simulink library "Libs_second"  (R2023b)
settings: Solver=VariableStepAuto  StartTime=0.0  StopTime=10.0  RelTol=1e-3
libraries: $bdroot x3, simulink x1
(part 2 of 2)

== stateflow chart Libs_second/Node_N_V6/Automaton ==
  settings: updateMethod=DISCRETE  executeAtInitialization=1
  state PacemakerCell
    state Cell [parallel]
      settings: executionOrder=1
      state Slow
        en: q=1; %phase4
      state Stimulated
        en: q=2; %phase0
        f1theta=exp(-h*theta);
        Vmax=(-1)*MDP*f1theta;
        [f3theta,n,Vmin]=sat(n,hr,hs,Vh1,s,m,theta);
      state Plateau
        en: q=3;%phase2
      state RP
        en:q=0;%phase3
      (default) -> Slow : /{Vmin=0;Vmax=(-1)*MDP; d3=d3fcn(MDP,VR,VT,d0,d2,ERP); BCL=RR(BCLin,SDin,f1in,f2in,sigma1sqin,sigma2sqin,t);...
          | t3=(abs(MDP)-VR)/abs(d3); t0=VR/abs(d0);t2=(abs(MDP)-VT)/abs(d2);d1=(VT)/(BCL-t3-t0-t2);d1out=d1;}
      Slow -> Stimulated [order 1] : [gv>VT&& v<VT]{theta=(v-VT)/(Vmin-VT);f2theta=exp(-f*theta);d2out=d2*f2theta;...
          |  f4theta=exp(j*(theta-1)); Vh1=Vh*f4theta; n=n+1;  ...
          |  vreset=v;reset; }
      Slow -> Stimulated [order 2] : [v>=VT]{theta=0; f2theta=exp(-f*theta); d2out=d2*f2theta;...
          |  n=(1-r)*n;  vreset=v;reset; }
      RP -> Slow : [v<=Vmin]{t3=(abs(MDP)-VR)/abs(d3); t0=VR/abs(d0);...
          | MDP=MDPin; VT=VTin; d2=d2in; t2=(abs(MDP)-VT)/abs(d2);...
          | BCL=RR(BCLin,SDin,f1in,f2in,sigma1sqin,sigma2sqin,t);...
          | d1=(VT)/(BCL-t3-t0-t2); d1out=d1*f3theta;...
          | VR=VRin; h=hin; Vh=Vhin; hs=hsin; r=rin;hr=hrin;d0=d0in;...
          | s=sin; j=jin; m=mm; ERP=ERPin;f=fin;...
          | vreset=v;reset;}
      Stimulated -> Plateau : [v>=Vmax]{d3=d3fcn(MDP,VR,VT,d0,d2,ERP);...
          | d3out=d3*f2theta;...
          | vreset=v;reset;}
      Plateau -> RP : [v<=VR]{d0out=d0*f2theta; vreset=v;reset;}
    state R [parallel]
      du:
      t=temporalCount(sec);
      settings: executionOrder=2
  (default) -> PacemakerCell : {t=0; MDP=MDPin;VT=VTin;VR=VRin;h=hin;Vh=Vhin;hs=hsin;r=rin;hr=hrin;d2=d2in;d0=d0in;...
      | s=sin;j=jin;m=mm;ERP=ERPin;f=fin;}
  data: f3out function_output double; tout function_output double; pt function_input double; Vminout function_output double; phr function_input double; phs function_input double; pVh function_input double; ps function_input double; pm function_input double; ptheta function_input double; pbcl function_input double; psd function_input double; pf1 function_input double; pf2 function_input double; psigma1sq function_input double; psigma2sq function_input double; rr function_output double size=1; pt function_input double; pMDP function_input double; pVR function_input double; pVT function_input double; pd0 function_input double; pd2 function_input double; pERP function_input double; d3in function_output double; q output double; MDPin input double =0; VTin input double; VRin input; Vmax local double; theta output double; vreset output double; gv input; v input double; hin input double; f1theta local double; Vhin input double; Vh1 local double; hsin input double; rin input double; hrin input double; Vmin local double; d2in input double; d3out output double; d0in input double; BCLin input double; SDin input double; f1in input double; f2in input double; sigma1sqin input double; sigma2sqin input double; d1out output double; Vtemp local double; t local double; sin input double; jin input double; mm input double; ERPin input double; f3theta local double; d2out output double; fin input double; d0out output double; f2theta local double; n local double; f4theta local double; d2 local double; Vh local double; h local double; hr local double; hs local double; j local double; m local double; r local double; s local double; BCL local double; ERP local double; MDP local double; VR local double; VT local double; d0 local double; f local double; d1 local double; d3 local double; t0 local double; t2 local double; t3 local double
  data v settings: updateMethod=SF_CONTINUOUS_TIME_DATA
  events: reset output EITHER_EDGE_EVENT
  function [f3out,tout,Vminout]=sat(pt,phr,phs,pVh,ps,pm,ptheta):
    | function [f3out,tout,Vminout]=sat(pt,phr,phs,pVh,ps,pm,ptheta)
    | 
    | td=phr*(pt-phs);
    | 
    | if td>=5
    |     tout=5/phr+phs;
    | else
    |     tout=pt;
    | end
    | 
    | if tout<1
    | co=0;
    | else
    | Vtemp=1+exp(-phr*(tout-phs)); 
    | co=1/Vtemp;
    | end;
    | Vminout=pVh*co;
    | thetai=ptheta;
    | for i=1:ps-1
    |     thetai=thetai*ptheta;
    | end
    | ft=pm*co*thetai+1;
    | f3out=1/ft;
    | end
  function rr= RR(pbcl,psd,pf1,pf2,psigma1sq,psigma2sq,pt):
    | function rr= RR(pbcl,psd,pf1,pf2,psigma1sq,psigma2sq,pt)
    | %Rate dependent factor
    | c1=0.01;
    | c2=0.01;
    | if psigma1sq<0 || psigma2sq<0
    |     error('Invalid input');
    | end
    | % The Gaussian frequency distribution, power spectrum
    | hf=0.5;
    | fstep=0.025;
    | ff=0:fstep:hf; % The frequency range original;
    | % fmax=1; % Assume the highest frequency
    | % fmin=0.025; % Assume the lowest frequency
    | % Fs=2*fmax; % The sample frequency 
    | % tstep=1/Fs; % The sample period of the time series
    | % tmax=1/fmin; % The period of the time series
    | % N=tmax/tstep;
    | % fstep=2*fmax/N; % =fmin
    | % f=fstep:fstep:fmax; % The frequency range original; 
    | ln=length(ff); % The number of frequency/cos signals.
    | s1=(psigma1sq/(c1*sqrt(2*pi)))*exp(-(ff-pf1).^2/(2*c1^2));
    | s2=(psigma2sq/(c2*sqrt(2*pi)))*exp(-(ff-pf2).^2/(2*c2^2));
    | ss=s1+s2; % s(f)
    | rss=sqrt(ss); %
    | %Construct the time series y(t) from s(f);
    | mag=rss; % the amplitudes;
    | y = ff'*2*pi*pt;
    | y = cos(y);
    | for i=1:ln
    |     y(i,:)=y(i,:)*mag(i);
    | end
    | if ln>1
    |     y1=sum(y);
    | else
    |     y1=y;
    | end
    | rr=pbcl+y1*psd;
    | end
  function d3in= d3fcn(pMDP,pVR,pVT,pd0,pd2,pERP):
    | function d3in= d3fcn(pMDP,pVR,pVT,pd0,pd2,pERP)
    | %#codegen
    | d3in=-(abs(pMDP)-pVR)/(pERP-(abs(pMDP)-pVT)/pd2-pVR/abs(pd0));

== stateflow chart Libs_second/Path_V3/Path ==
  settings: updateMethod=DISCRETE
  state Wave
    state Relay_i [parallel]
      settings: executionOrder=8
      state Relay
        en: tj_1=0;
        du: tj_1=temporalCount(sec);
        vj_1=vbi(floor(tj_1)+1);
        ex: tj_1=0;
      state Idle
        en:
        vj_1=0;
      Wave.Relay_i.Idle -> Wave.Relay_i.Relay : Reach_j
      (default) -> Wave.Relay_i.Idle
      Wave.Relay_i.Relay -> Wave.Relay_i.Idle : [qj>=2 || j_1==0 ]
    state Cell_i_1 [parallel]
      settings: executionOrder=5
      state Activation
      state Rest
        en:
        i_1=0;
      Wave.Cell_i_1.Rest -> Wave.Cell_i_1.Activation : Reach_i
      Wave.Cell_i_1.Activation -> Wave.Cell_i_1.Rest [order 1] : [after(tbj,sec)]
      (default) -> Wave.Cell_i_1.Rest
      Wave.Cell_i_1.Activation -> Wave.Cell_i_1.Rest [order 2] : Go_j
    state Relay_j [parallel]
      settings: executionOrder=7
      state Relay
        en: ti_1=0;
        du: ti_1=temporalCount(sec);
        vi_1=vbj(floor(ti_1)+1);
        ex: ti_1=0;
      state Idle
        en:
        vi_1=0;
      Wave.Relay_j.Idle -> Wave.Relay_j.Relay : Reach_i
      (default) -> Wave.Relay_j.Idle
      Wave.Relay_j.Relay -> Wave.Relay_j.Idle : [qi>=2 || i_1==0 ]
    state Cell_j_1 [parallel]
      settings: executionOrder=6
      state Activation
      state Rest
        en:
        j_1=0;
      note: 1.
      Wave.Cell_j_1.Rest -> Wave.Cell_j_1.Activation : Reach_j
      Wave.Cell_j_1.Activation -> Wave.Cell_j_1.Rest [order 1] : [after(tbi,sec)]
      (default) -> Wave.Cell_j_1.Rest
      Wave.Cell_j_1.Activation -> Wave.Cell_j_1.Rest [order 2] : Go_i
    state End_j [parallel]
      settings: executionOrder=2
      state End_j_Idle
      state Go
        en: tj=0;
        du: tj=temporalCount(sec);
        ex: tj=0;
      note: 5
      state Ready
      note: 2.
      state BlockedByNeighbour
      Wave.End_j.Go -> Wave.End_j.End_j_Idle [order 2] : [Meet || mul==0]
      Wave.End_j.Go -> Wave.End_j.End_j_Idle [order 1] : [tj>=Tj && mul==1]
          | /{mul=mul-1;i_1=1; Reach_i;}
      (default) -> Wave.End_j.End_j_Idle
      Wave.End_j.End_j_Idle -> Wave.End_j.Ready [order 1] : [qj==2 && j_1==0]
      Wave.End_j.Ready -> Wave.End_j.Go [order 2] : [qj==3 && j_1==0]
          | /{ cvj=thetafcn(cvji,thetaj,aji,bji,cji);
          | Tj=l/cvj; mul=mul+1; Go_j;}
      Wave.End_j.End_j_Idle -> Wave.End_j.BlockedByNeighbour [order 2] : [qj==2 && j_1==1]
      Wave.End_j.Ready -> Wave.End_j.BlockedByNeighbour [order 1] : [cvji==0 || (qj==3 && j_1==1)]{tj=0;}
      Wave.End_j.BlockedByNeighbour -> Wave.End_j.End_j_Idle : [qj==0]
    state End_i [parallel]
      settings: executionOrder=1
      state Go
        en:ti=0;
        du: ti=temporalCount(sec);
        ex: ti=0;
      state End_i_Idle
      note: 4
      state Ready
      note: 2.
      note: 7
      state BlockedByNeighbour
      Wave.End_i.Go -> Wave.End_i.End_i_Idle [order 2] : [cvi*ti+cvj*tj>=l && mul==2]/
          | { mul=0; Meet;}
      Wave.End_i.Go -> Wave.End_i.End_i_Idle [order 1] : [ti>=Ti && mul==1]
          | /{mul=mul-1; j_1=1; Reach_j;}
      (default) -> Wave.End_i.End_i_Idle
      Wave.End_i.End_i_Idle -> Wave.End_i.Ready [order 1] : [qi==2 && i_1==0]
      Wave.End_i.Ready -> Wave.End_i.Go [order 2] : [qi==3 && i_1==0]
          | /{ cvi=thetafcn(cvij,thetai,aij,bij,cij);
          | Ti=l/cvi; mul=mul+1;Go_i; }
      Wave.End_i.End_i_Idle -> Wave.End_i.BlockedByNeighbour [order 2] : [qi==2 && i_1==1]
      Wave.End_i.Ready -> Wave.End_i.BlockedByNeighbour [order 1] : [cvij==0 || (qi==3 && i_1==1)]{ti=0;}
      Wave.End_i.BlockedByNeighbour -> Wave.End_i.End_i_Idle : [qi==0]
    state Buffer_i [parallel]
      settings: executionOrder=3
      state Idle
      note: 6
      state Buffer_i
        en: tbi=0;
        du: tbi=temporalCount(sec);
        vbi(floor(tbi)+1)=vi;
      (default) -> Wave.Buffer_i.Idle
      Wave.Buffer_i.Idle -> Wave.Buffer_i.Buffer_i : Go_i
      Wave.Buffer_i.Buffer_i -> Wave.Buffer_i.Idle [order 1] : [qi<3]
      Wave.Buffer_i.Buffer_i -> Wave.Buffer_i.Idle [order 2] : Meet
      Wave.Buffer_i.Buffer_i -> Wave.Buffer_i.Idle [order 3] : [tbi>=0.599]
    note: 3
    state Buffer_j [parallel]
      settings: executionOrder=4
      state Idle
      state Buffer_i
        en: tbj=0;
        du: tbj=temporalCount(sec);
        vbj(floor(tbj)+1)=vj;
      (default) -> Wave.Buffer_j.Idle
      Wave.Buffer_j.Idle -> Wave.Buffer_j.Buffer_i : Go_j
      Wave.Buffer_j.Buffer_i -> Wave.Buffer_j.Idle [order 1] : [qj<3]
      Wave.Buffer_j.Buffer_i -> Wave.Buffer_j.Idle [order 2] : Meet
      Wave.Buffer_j.Buffer_i -> Wave.Buffer_j.Idle [order 3] : [tbj>=0.599]
    state End_i_Fade [parallel]
      settings: executionOrder=10
      state End_i_Idle
      state End_i_re
        du: tir=temporalCount(sec);
      End_i_re -> Wave.End_i_Fade.End_i_Idle [order 1] : [cvi*tir+cvj*tjr>=l && tjr~=0]/{Meet_r;tir=0;tjr=0;}
      End_i_re -> Wave.End_i_Fade.End_i_Idle [order 2] : [cvi*tir+cvj*tjr>=l&& tjr==0]/{tir=0;}
      (default) -> Wave.End_i_Fade.End_i_Idle
      Wave.End_i_Fade.End_i_Idle -> End_i_re : cell_i_r
    state End_j_Fade [parallel]
      settings: executionOrder=12
      state End_j_Idle
      state End_j_re
        du: tjr=temporalCount(sec);
      End_j_re -> Wave.End_j_Fade.End_j_Idle [order 1] : [cvi*tir+cvj*tjr>=l&& tir==0]/{tjr=0;}
      End_j_re -> Wave.End_j_Fade.End_j_Idle [order 2] : Meet_r
      (default) -> Wave.End_j_Fade.End_j_Idle
      Wave.End_j_Fade.End_j_Idle -> End_j_re : cell_j_r
    state Celll_j_Re [parallel]
      settings: executionOrder=9
      state Re
      state De
      Wave.Celll_j_Re.De -> Wave.Celll_j_Re.Re : [qj==0]/{cell_j_r;}
      Wave.Celll_j_Re.Re -> Wave.Celll_j_Re.De : [qj==3]
      (default) -> Wave.Celll_j_Re.Re
    state Celll_i_Re [parallel]
      settings: executionOrder=11
      state Re
      state De
      Wave.Celll_i_Re.De -> Wave.Celll_i_Re.Re : [qi==0]/{cell_i_r;}
      Wave.Celll_i_Re.Re -> Wave.Celll_i_Re.De : [qi==3]
      (default) -> Wave.Celll_i_Re.Re
    note: 1. The Cell_j_1 will be released if it has been resting or another AP from Cell_i starts travelling;.
    note: 2. Cell_i start to repolarize before the activation either reaches Cell_j or meets the activation from Cell_j, which happens when the APD is short or/and the path is long, e.g., premature depolarization.
        | In this case, the path would ignore all following activation before the premature activation reaches Cell_j or meets the activation from Cell_j.
  note: 3. Assume that the APD<=600 ms; If the APD>600, it would be truncated; Store the action potential of q3 until it goes back to repolarization or meets the other one.
      | 4. j_1=1; and Reach_j must occur at the same time to block Go_j immediately;
      | 5. mul==0 to make sure the transition to take in case Meet event is missed
      | 6. qi<3 instead of qi==0 to avoid where qi==0 is missed due to the stimulation timing and the simulation step;
      | 7. when cv=0, no propagation.
  (default) -> Wave : /{l=sqrt((xj-xi)^2+(yj-yi)^2);
      | cvi=cvij;
      | cvj=cvji;
      | Ti=1/cvi;
      | Tj=1/cvj;
      | ti=0;
      | tj=0;
      | ti_1=0;
      | tj_1=0;
      | i_1=0;
      | j_1=0;
      | vi_1=0;
      | vj_1=0;
      | tir=0;
      | tjr=0;
      | tbi=0;
      | tbj=0;
      | vbi=zeros(1,600);
      | vbj=zeros(1,600);
      | mul=0;
      | }
  data: cvin function_input double; thetain function_input double; ain function_input double; bin function_input double; cin function_input double; cvout function_output double; cvi output double; cvj output double; ti output double; qi input; qj input; ti_1 local double; tj_1 local double; cvij input; thetai input; aij input; bij input; cij input; cvji input; thetaj input; aji input; bji input; cji input; xi input; yi input; xj input; yj input; tj output; tir output; tjr output; i_1 local; j_1 local; vi_1 output; vj_1 output; l local; tbi local; tbj local; vbi local; vbj local; vi input; vj input; Ti local double; Tj local double; mul local
  events: Reach_i local FUNCTION_CALL_EVENT; Reach_j local FUNCTION_CALL_EVENT; Go_i local FUNCTION_CALL_EVENT; Go_j local FUNCTION_CALL_EVENT; Meet local FUNCTION_CALL_EVENT; Meet_r local FUNCTION_CALL_EVENT; cell_i_r local FUNCTION_CALL_EVENT; cell_j_r local FUNCTION_CALL_EVENT
  function cvout = thetafcn(cvin,thetain,ain,bin,cin):
    | function cvout = thetafcn(cvin,thetain,ain,bin,cin)
    | %#codegen
    | %Rate dependent factor
    | ftheta=1/(ain*exp(bin*thetain)+(1-ain)*exp(-cin*thetain));
    | cvout=cvin*ftheta;
    | end

== stateflow chart Libs_second/PM_DDD_v3/DDD ==
  state DDD
    state AVI [parallel]
      settings: executionOrder=1
      state st1
      state st2
      state st3
      state st3C_CC
      st1 -> st2 : a_p||a_s[(sent~=-1)]/{n_t=0;}
      st2 -> st1 [order 3] : v_s[(sent~=-1)]/{}
      st2 -> st1 [order 2] : [(sent==0)&&(comm==0)&&(URIex==1)&&(temporalCount(clk)==AVId-n_t)]/{sent=3;}
      st3 -> st1 [order 1] : v_s[(sent~=-1)]/{}
      (default) -> st1
      st3C_CC -> st1 : [(sent==0)]/{sent=3;comm=comm-1;act=1;}
      st2 -> st3 [order 1] : [(sent==0)&&(comm==0)&&(URIex==0)&&(temporalCount(clk)==AVId-n_t)]/{}
      st3 -> st3C_CC [order 2] : uri_s[(sent~=-1)]/{comm=comm+1;act=1;}
    state LRI [parallel]
      settings: executionOrder=2
      state LRI
      state LRI_AS
      (default) -> DDD.LRI.LRI
      DDD.LRI.LRI -> DDD.LRI.LRI [order 1] : [(sent==0)&&(comm==0)&&(temporalCount(clk)==LRId-AVId-n_t)]
          | /{sent=1;n_t=0;}
      DDD.LRI.LRI -> LRI_AS [order 3] : a_s[(sent~=-2)]/{}
      LRI_AS -> DDD.LRI.LRI : v_p||v_s[(sent~=-2)]/{n_t=0;}
      DDD.LRI.LRI -> DDD.LRI.LRI [order 2] : v_p||v_s[(sent~=-2)]/{n_t=0;}
    state URI [parallel]
      settings: executionOrder=5
      state URIst2
      state URIst1
      (default) -> URIst1
      URIst1 -> URIst2 [order 2] : [(sent==0)&&(comm==0)&&(temporalCount(clk)==URId-n_t)]
          | /{sent=9;act=1;URIex=1;}
      URIst2 -> URIst1 : v_p||v_s[(sent~=-5)]/{n_t=0;act=1;URIex=0;}
      URIst1 -> URIst1 [order 1] : v_p||v_s[(sent~=-5)]/{n_t=0;}
    state PVARP [parallel]
      settings: executionOrder=3
      state ARPst1
      state ARPst2
      state AB
      state inter_CC
      ARPst2 -> ARPst1 [order 1] : [(sent==0)&&(comm==0)&&(temporalCount(clk)==PVARPd-n_t)]/{}
      (default) -> ARPst1
      ARPst1 -> ARPst2 [order 1] : v_p||v_s[(sent~=-3)]/{n_t=0;}
      AB -> ARPst2 : v_p||v_s[(sent~=-3)]/{n_t=0;}
      ARPst2 -> ARPst2 [order 2] : v_p||v_s[(sent~=-3)]/{n_t=0;}
      ARPst1 -> AB [order 3] : a_p[(sent~=-3)]/{n_t=0;}
      ARPst1 -> DDD.PVARP.inter_CC [order 2] : [AinB==1 &&(sent~=-3)]
          | /{comm=comm+1;
          | act=1;}
      DDD.PVARP.inter_CC -> AB : [(sent==0)]/{sent=2;comm=comm-1;act=1;}
    state VRP [parallel]
      settings: executionOrder=4
      state VRPst1
      state VRPst2
      state inter_CC
      VRPst2 -> VRPst1 : [(sent==0)&&(comm==0)&&(temporalCount(clk)==VRPd-n_t)]/{}
      (default) -> VRPst1
      VRPst1 -> VRPst2 [order 2] : v_p[(sent~=-4)]/{n_t=0;}
      DDD.VRP.inter_CC -> VRPst2 : [(sent==0)]/{sent=4;n_t=0;comm=comm-1;act=1;}
      VRPst1 -> DDD.VRP.inter_CC [order 1] : [VinB==1&&(sent~=-4)]
          | /{n_t=0;comm=comm+1;
          | act=1;}
    state Eng [parallel]
      settings: executionOrder=6
      state E
      note: Reactivate the chart
          | to allow more than one transitions occur
          | during a clk execution
      (default) -> E
      E -> E [order 2] : [sent==4]{sent=-4;send(v_s);}/{VS;}
      E -> E [order 6] : [sent==3]{sent=-1;send(v_p);}/{VP;}
      E -> E [order 3] : [sent==9]{sent=-5;send(uri_s);}
      E -> E [order 5] : [sent==2]{sent=-3;send(a_s);}/{AS;}
      E -> E [order 1] : [sent<0]{sent=0;send(tt);}
      E -> E [order 4] : [sent==1]{sent=-2;send(a_p);}/{AP;}
      E -> E [order 7] : [act==1]{act=0;send(tt);}
  note: [(sent==0] disables all "non-receiving "
  note: [(sent~=-*] disables all "receiving "
  note: add Atrial blanking
  data: LRId input; sent local int8; n_t local double; act local boolean; comm local double; AVId input; URId input; VRPd input; URIex local boolean; PVARPd input; AinB input double; VinB input double
  events: a_p local FUNCTION_CALL_EVENT; a_s local FUNCTION_CALL_EVENT; v_p local FUNCTION_CALL_EVENT; v_s local FUNCTION_CALL_EVENT; AP output EITHER_EDGE_EVENT; clk input RISING_EDGE_EVENT; uri_s local FUNCTION_CALL_EVENT; tt local FUNCTION_CALL_EVENT; VP output EITHER_EDGE_EVENT; AS output EITHER_EDGE_EVENT; VS output EITHER_EDGE_EVENT

== stateflow chart Libs_second/PM_DDD_v3/pul ==
  settings: executeAtInitialization=1
  state width
  state Ini
    en:
    eve=0;
  Ini -> width : event{eve=1;}
  (default) -> Ini
  width -> Ini : [after(2,clk)]
  data: eve output
  events: clk input RISING_EDGE_EVENT; event input EITHER_EDGE_EVENT

== stateflow chart Libs_second/PM_DDD_v3/pul1 ==
  settings: executeAtInitialization=1
  state width
  state Ini
    en:
    eve=0;
  Ini -> width : event{eve=1;}
  (default) -> Ini
  width -> Ini : [after(2,clk)]
  data: eve output
  events: clk input RISING_EDGE_EVENT; event input EITHER_EDGE_EVENT

== stateflow chart Libs_second/PM_DDD_v3/pul2 ==
  settings: executeAtInitialization=1
  state width
  state Ini
    en:
    eve=0;
  Ini -> width : event{eve=1;}
  (default) -> Ini
  width -> Ini : [after(2,clk)]
  data: eve output
  events: clk input RISING_EDGE_EVENT; event input EITHER_EDGE_EVENT

== stateflow chart Libs_second/PM_DDD_v3/pul3 ==
  settings: executeAtInitialization=1
  state width
  state Ini
    en:
    eve=0;
  Ini -> width : event{eve=1;}
  (default) -> Ini
  width -> Ini : [after(2,clk)]
  data: eve output
  events: clk input RISING_EDGE_EVENT; event input EITHER_EDGE_EVENT

== stateflow chart Libs_second/Cnds_DDDv1/pps ==
  state M
    state AVI [parallel]
      settings: executionOrder=4
      state Idle
      state AVI
        en:
        tv4=0;
        du:
        tv4=temporalCount(sec);
      (default) -> M.AVI.Idle
      M.AVI.Idle -> M.AVI.AVI : AS||AP
      M.AVI.AVI -> M.AVI.Idle [order 1] : VS[tv4<=AVI+a]{RegPP(18);ps=ps+1;allps(1,ps)=t;...
          | allps(2,ps)=tv4;allps(3,ps)=18;}
      M.AVI.AVI -> M.AVI.Idle [order 2] : VP[tv4<AVI-a&&tv4>a]{RegPP(19);ps=ps+1;allps(1,ps)=t;...
          | allps(2,ps)=tv4;allps(3,ps)=19;errn=errn+1;errs(1,errn)=t;...
          | errs(2,errn)=tv4;errs(3,errn)=7;}
      M.AVI.AVI -> M.AVI.AVI [order 10] : AS[tv4>a]{RegPP(27);ps=ps+1;allps(1,ps)=t;...
          | allps(2,ps)=tv4;allps(3,ps)=27;}
      M.AVI.AVI -> M.AVI.Idle [order 3] : VP[tv4>=AVI-a &&tv4<=AVI+a&&tv<URI-a]{RegPP(20);ps=ps+1;allps(1,ps)=t;...
          | allps(2,ps)=tv4;allps(3,ps)=20;errn=errn+1;errs(1,errn)=t;...
          | errs(2,errn)=tv4;errs(3,errn)=8;}
      M.AVI.AVI -> M.AVI.AVI [order 12] : AS||AP[tv4<=a]
      M.AVI.AVI -> M.AVI.Idle [order 4] : VP[tv4>=AVI-a &&tv4<=AVI+a&&tv>=URI-a]{RegPP(21);ps=ps+1;allps(1,ps)=t;...
          | allps(2,ps)=tv4;allps(3,ps)=21;}
      M.AVI.AVI -> M.AVI.Idle [order 5] : VP[tv4>AVI+a&&tv<URI-a]{RegPP(22);ps=ps+1;allps(1,ps)=t;...
          | allps(2,ps)=tv4;allps(3,ps)=22;errn=errn+1;errs(1,errn)=t;...
          | errs(2,errn)=tv4;errs(3,errn)=9;}
      M.AVI.AVI -> M.AVI.Idle [order 6] : VP[tv4>AVI+a&&tv>=URI-a &&tv<=URI+a]{RegPP(23);ps=ps+1;allps(1,ps)=t;...
          | allps(2,ps)=tv4;allps(3,ps)=23;}
      M.AVI.AVI -> M.AVI.AVI [order 11] : AP[tv4>a]{RegPP(28);ps=ps+1;allps(1,ps)=t;...
          | allps(2,ps)=tv4;allps(3,ps)=28;...
          | errn=errn+1;errs(1,errn)=t;...
          | errs(2,errn)=tv4;errs(3,errn)=12;}
      M.AVI.AVI -> M.AVI.Idle [order 7] : VP[tv4>AVI+a&&tv>URI+a]{RegPP(24);ps=ps+1;allps(1,ps)=t;...
          | allps(2,ps)=tv4;allps(3,ps)=24;errn=errn+1;errs(1,errn)=t;...
          | errs(2,errn)=tv4;errs(3,errn)=10;}
      M.AVI.AVI -> M.AVI.Idle [order 8] : VS[tv4>AVI+a&&tv<=URI+a]{RegPP(25);ps=ps+1;allps(1,ps)=t;...
          | allps(2,ps)=tv4;allps(3,ps)=25;}
      M.AVI.AVI -> M.AVI.Idle [order 9] : VS[tv4>AVI+a&&tv>URI+a]{RegPP(26);ps=ps+1;allps(1,ps)=t;...
          | allps(2,ps)=tv4;allps(3,ps)=26;errn=errn+1;errs(1,errn)=t;...
          | errs(2,errn)=tv4;errs(3,errn)=11;}
      M.AVI.AVI -> M.AVI.Idle [order 13] : VP[tv4<=a]
    note: allpp=[req1,req2,req3,req4,frequency]
        | allps=[t, t', req]';
        | errs=[t, t',err]'
    state LRI [parallel]
      settings: executionOrder=3
      state Idle
      state AEI
        en:
        tv3=0;
        du:
        tv3=temporalCount(sec);
      (default) -> M.LRI.Idle
      AEI -> AEI [order 6] : VS[tv3>a]{RegPP(16);ps=ps+1;allps(1,ps)=t;...
          | allps(2,ps)=tv3;allps(3,ps)=16;}
      M.LRI.Idle -> AEI : VS||VP
      AEI -> M.LRI.Idle [order 1] : AS[tv3<=AEI+a]{RegPP(11);ps=ps+1;allps(1,ps)=t;...
          | allps(2,ps)=tv3;allps(3,ps)=11;}
      AEI -> AEI [order 8] : VS||VP[tv3<=a]
      AEI -> M.LRI.Idle [order 2] : AP[tv3<AEI-a&&tv3>a]{RegPP(12);ps=ps+1;allps(1,ps)=t;...
          | allps(2,ps)=tv3;allps(3,ps)=12;errn=errn+1;errs(1,errn)=t;...
          | errs(2,errn)=tv3;errs(3,errn)=3;}
      AEI -> M.LRI.Idle [order 3] : AP[tv3>=AEI-a && tv3<=AEI+a]{RegPP(13);ps=ps+1;allps(1,ps)=t;...
          | allps(2,ps)=tv3;allps(3,ps)=13;}
      AEI -> AEI [order 7] : VP[tv3>a]{RegPP(17);ps=ps+1;allps(1,ps)=t;...
          | allps(2,ps)=tv3;allps(3,ps)=17;errn=errn+1;errs(1,errn)=t;...
          | errs(2,errn)=tv3;errs(3,errn)=6;}
      AEI -> M.LRI.Idle [order 4] : AP[tv3>AEI+a]{RegPP(14);ps=ps+1;allps(1,ps)=t;...
          | allps(2,ps)=tv3;allps(3,ps)=14;errn=errn+1;errs(1,errn)=t;...
          | errs(2,errn)=tv3;errs(3,errn)=4;}
      AEI -> M.LRI.Idle [order 5] : AS[tv3>AEI+a]{RegPP(15);ps=ps+1;allps(1,ps)=t;...
          | allps(2,ps)=tv3;allps(3,ps)=15;errn=errn+1;errs(1,errn)=t;...
          | errs(2,errn)=tv3;errs(3,errn)=5;}
      AEI -> M.LRI.Idle [order 9] : AP[tv3<=a]
    state URI [parallel]
      settings: executionOrder=5
      state Timing
        en:
        tv=0;
        du:
        tv=temporalCount(sec);
      state wait
      (default) -> wait
      Timing -> Timing : VS||VP
      wait -> Timing : VS||VP
    state PVAsense [parallel]
      settings: executionOrder=2
      state WaitV
      state PVARP
        en:
        tv2=0;
        du:
        tv2=temporalCount(sec);
      state Out_PVARP
        en:
        tv2=PVARP;
        du:
        tv2=PVARP+temporalCount(sec);
      state Idle
      PVARP -> PVARP [order 2] : VP||VS
      WaitV -> PVARP : VS||VP
      PVARP -> WaitV [order 1] : AS[tv2>=PVARP-a && tv2<=PVARP+a]
          | {RegPP(9);ps=ps+1;allps(1,ps)=t;...
          | allps(2,ps)=tv2;allps(3,ps)=9;}
      (default) -> M.PVAsense.Idle
      PVARP -> Out_PVARP [order 3] : [tv2>=PVARP+a]
      PVARP -> WaitV [order 4] : AS[tv2<PVARP-a]
          | {RegPP(10);ps=ps+1;allps(1,ps)=t;...
          | allps(2,ps)=tv2;allps(3,ps)=10;...
          | errn=errn+1;errs(1,errn)=t;...
          | errs(2,errn)=tv2;errs(3,errn)=2;}
      M.PVAsense.Idle -> WaitV [order 1] : AS{RegPP(7);ps=ps+1;allps(1,ps)=t;...
          | allps(2,ps)=tv2;allps(3,ps)=7;}
      Out_PVARP -> PVARP [order 1] : VS||VP
      M.PVAsense.Idle -> WaitV [order 2] : AP{RegPP(6);ps=ps+1;allps(1,ps)=t;...
          | allps(2,ps)=tv2;allps(3,ps)=6;}
      Out_PVARP -> WaitV [order 2] : AS{RegPP(9);ps=ps+1;allps(1,ps)=t;...
          | allps(2,ps)=tv2;allps(3,ps)=9;}
      Out_PVARP -> WaitV [order 3] : AP{RegPP(8);ps=ps+1;allps(1,ps)=t;...
          | allps(2,ps)=tv2;allps(3,ps)=8;}
    state Vsense [parallel]
      settings: executionOrder=1
      state VRP
        en:
        tv1=0;
        du:
        tv1=temporalCount(sec);
      state Out_VRP
      state Idle
      VRP -> VRP [order 1] : VS[tv1>=VRP-a && tv1<=VRP+a]{RegPP(3);ps=ps+1;allps(1,ps)=t;...
          | allps(2,ps)=tv1;allps(3,ps)=3;}
      (default) -> M.Vsense.Idle
      M.Vsense.Idle -> VRP [order 2] : VP{RegPP(2);ps=ps+1;allps(1,ps)=t;...
          | allps(2,ps)=tv1;allps(3,ps)=2;}
      VRP -> Out_VRP [order 3] : [tv1>=VRP+a]
      M.Vsense.Idle -> VRP [order 1] : VS{RegPP(1);ps=ps+1;allps(1,ps)=t;...
          | allps(2,ps)=tv1;allps(3,ps)=1;}
      Out_VRP -> VRP [order 1] : VS{RegPP(3);ps=ps+1;allps(1,ps)=t;...
          | allps(2,ps)=tv1;allps(3,ps)=3;}
      VRP -> VRP [order 2] : VP
      Out_VRP -> VRP [order 2] : VP{RegPP(4);ps=ps+1;allps(1,ps)=t;...
          | allps(2,ps)=tv1;allps(3,ps)=4;}
      VRP -> VRP [order 4] : VS[tv1<VRP-a]{RegPP(5);ps=ps+1;allps(1,ps)=t;...
          | allps(2,ps)=tv1;allps(3,ps)=5;...
          | errn=errn+1;errs(1,errn)=t;...
          | errs(2,errn)=tv1;errs(3,errn)=1;}
  (default) -> M : { cov=zeros(1,5);...
      | allpp=zeros(150,5);...
      | allps=zeros(3,300);...
      | errs=zeros(3,300);...
      | N= 0; len= 0; ps=0; ...
      | errn=0;...
      | tv=URI;a=3; ...
      | AEI=LRI-AVI;...
      | tv1=0;
      | tv2=0;
      | tv3=0;
      | tv4=0;}
  data: element function_input; VRP input; PVARP input; LRI input; URI input; tv1 local double; tv2 local double; tv3 local double; tv4 local double; AVI input; cov local double size=[1 5]; len local double; N output double; allpp output double size=[150 5]; errn output double; errs output double size=[3 300]; allps output double size=[3 300]; ps local double; a local double; t input; AEI local double; tv local double
  events: clk input RISING_EDGE_EVENT; AS input RISING_EDGE_EVENT; AP input RISING_EDGE_EVENT; VS input RISING_EDGE_EVENT; VP input RISING_EDGE_EVENT
  function RegPP(element):
    | %% Get the index of the parameter
    | function RegPP(element)
    | %#codegen
    | coder.extrinsic('isequal');
    | npp=4;
    | % Put the element at the end of the queue
    | len=len+1;
    | cov(1,len)=element;
    | % The number of combination is 1 to the lenth of the queue when the
    | % queue is not full. 
    | if len<=npp
    |     N=1;
    |     allpp(1,1:npp)=cov(1:npp);
    | end
    | %Remove the front element of the queue and move the other elements forward
    | if len==npp+1
    |     for i=1:len-1
    |         cov(1,i)=cov(1,i+1);
    |     end
    |     cov(1,npp+1)=0;
    |     len=len-1;
    |     % To see if the combination has been tested
    |     temp=0;
    |     for j=1:N
    |         if isequal(cov(1:npp),allpp(j,1:npp))
    |             allpp(j,npp+1)=allpp(j,npp+1)+1;
    |             break
    |         end
    |         temp=temp+1;
    |     end
    |     if temp==N % This combination has not been tested
    |         N=N+1;
    |         allpp(N,1:npp)=cov(1:npp);
    |     end    
    | end
    | 
    | end

== stateflow chart Libs_second/Pre_eventsv1/Chart2 ==
  settings: executeAtInitialization=1
  state pulseout
  state Ini
  Ini -> pulseout : event{eve=1;}
  (default) -> Ini
  pulseout -> Ini : [temporalCount(clk)==2]{eve=0;}
  data: eve output
  events: clk input RISING_EDGE_EVENT; event input EITHER_EDGE_EVENT

== stateflow chart Libs_second/Pre_eventsv1/Chart1 ==
  settings: executeAtInitialization=1
  state pulseout
  state Ini
  Ini -> pulseout : event{eve=1;}
  (default) -> Ini
  pulseout -> Ini : [temporalCount(clk)==2]{eve=0;}
  data: eve output
  events: clk input RISING_EDGE_EVENT; event input EITHER_EDGE_EVENT

== stateflow chart Libs_second/PMTv1/PMT detection ==
  settings: executeAtInitialization=1
  state WaitVP
  state WaitAS
    en:
    t=0;
    du:
    t=temporalCount(clk);
  state Idle
  state PMT
  state RST
  WaitAS -> WaitVP [order 1] : AS[t<400]{s=s+1;}
  Idle -> WaitAS : VP{s=0;}
  (default) -> Idle
  WaitVP -> PMT [order 1] : [s==9]
  WaitVP -> WaitAS [order 2] : VP[s<9]
  WaitVP -> RST [order 3] : VS||AP||AS[s<9]
  WaitAS -> RST [order 2] : AS[t>=400]
  WaitAS -> RST [order 3] : VS||VP||AP
  RST -> WaitAS : VP{s=0;}
  data: s output double; t local double
  events: clk input RISING_EDGE_EVENT; AS input RISING_EDGE_EVENT; VS input RISING_EDGE_EVENT; AP input RISING_EDGE_EVENT; VP input RISING_EDGE_EVENT

== stateflow chart Libs_second/Pre_eventsv1/Events detection ==
  settings: executeAtInitialization=1
  state M
    state Vsense [parallel]
      settings: executionOrder=1
      note: [1]
      state VRP
        en:
        tv1=0;
        du:
        tv1=temporalCount(clk);
      state Out_VRP
      state Idle
      note: 1st Vget
      VRP -> VRP [order 1] : [Vget==1 &&tv1==VRP]/{VS;vs;}
      M.Vsense.Idle -> VRP [order 2] : VP
      VRP -> Out_VRP [order 3] : [Vget==0&&tv1>=VRP]
      (default) -> M.Vsense.Idle
      M.Vsense.Idle -> VRP [order 1] : [Vget==1]/{VS;vs;}
      Out_VRP -> VRP [order 1] : [Vget==1]/{VS;vs;}
      VRP -> VRP [order 2] : VP
      Out_VRP -> VRP [order 2] : VP
    state PVAsense [parallel]
      settings: executionOrder=2
      state Idle
      state PVARP
        en:
        tv2=0;
        du:
        tv2=temporalCount(clk);
      state Out_PVARP
      state WaitV
      note: [1]
      (default) -> M.PVAsense.Idle
      M.PVAsense.Idle -> PVARP [order 3] : VP||VS
      PVARP -> PVARP [order 2] : VP||VS
      PVARP -> Out_PVARP [order 3] : [Aget==0&&tv2>=PVARP]
      M.PVAsense.Idle -> WaitV [order 1] : [Aget==1]
          | /{as;}
      WaitV -> PVARP : VS||VP
      Out_PVARP -> PVARP [order 1] : VS||VP
      PVARP -> WaitV [order 1] : [Aget==1 &&tv2==PVARP]
          | /{as;}
      M.PVAsense.Idle -> WaitV [order 2] : AP
      Out_PVARP -> WaitV [order 2] : [Aget==1]
          | /{as;}
      Out_PVARP -> WaitV [order 3] : AP
  note: [1] Make sure that VS emits at tv1==VRP if Vget is present
  (default) -> M
  data: PVARP input; VRP input; Aget input double; Vget input double; tv1 local double; tv2 local double
  events: clk input RISING_EDGE_EVENT; as output EITHER_EDGE_EVENT; vs output EITHER_EDGE_EVENT; AP input RISING_EDGE_EVENT; VP input RISING_EDGE_EVENT; VS local EITHER_EDGE_EVENT

== stateflow chart Libs_second/Ratesv1/rates ==
  settings: executeAtInitialization=1
  state M
    state Rate_AM [parallel]
      settings: executionOrder=1
      state In1
        en:
        ta=0;
        du:
        ta=temporalCount(sec);
      state In
      M.Rate_AM.In1 -> M.Rate_AM.In1 [order 1] : AS[ta>a]{nas=nas+1;rate_as(1,nas)=t; rate_as(2,nas)=60000/ta;}
      (default) -> M.Rate_AM.In
      M.Rate_AM.In -> M.Rate_AM.In1 : AS||AP
      M.Rate_AM.In1 -> M.Rate_AM.In1 [order 2] : AP[ta>a]{nap=nap+1;rate_ap(1,nap)=t; rate_ap(2,nap)=60000/ta;}
    state Rate_VM [parallel]
      settings: executionOrder=2
      state In1
        en:
        tv=0;
        du:
        tv=temporalCount(sec);
      state In
      (default) -> M.Rate_VM.In
      M.Rate_VM.In1 -> M.Rate_VM.In1 [order 1] : VS[tv>a]{nvs=nvs+1;rate_vs(1,nvs)=t; rate_vs(2,nvs)=60000/tv;}
      M.Rate_VM.In -> M.Rate_VM.In1 : VS||VP
      M.Rate_VM.In1 -> M.Rate_VM.In1 [order 2] : VP[tv>a]{nvp=nvp+1;rate_vp(1,nvp)=t; rate_vp(2,nvp)=60000/tv;}
  (default) -> M : {rate_as=zeros(2,100);...
      | rate_ap=zeros(2,100);...
      | rate_vs=zeros(2,100);...
      | rate_vp=zeros(2,100);...
      | nas=0;nvs=0;...
      | nap=0; nvp=0;...
      | ta=0;tv=0;a=3;}
  data: t input; nas output double; nap output double; nvs output double; nvp output double; rate_as output double; rate_ap output double; rate_vs output double; rate_vp output double; ta local double; tv local double; a local
  events: clk input RISING_EDGE_EVENT; AS input RISING_EDGE_EVENT; VS input RISING_EDGE_EVENT; AP input RISING_EDGE_EVENT; VP input RISING_EDGE_EVENT
